simulink model "baseline_validation"  (R2024b)
settings: Solver=ode45  StartTime=0  StopTime=0.1  MaxStep=1e-4  RelTol=1e-8  AbsTol=1e-10
model workspace (MAT data in the model file):
  F = 0.008
  J = 0.003
  L = 0.0085
  Rs = 0.2
  inputFrequency = 20
  loadTorque = 0
  p = 4
  psi = 0.175
  voltageAmplitude = 30
Description:
  | AFPM 等效集中参数、非凸极 PMSM plant 独立验证；不代表三维磁场或完整闭环控制。
settings Model: Creator=m1516  LastModifiedBy=m1516
settings DataIOCC: SaveOutput=off  SignalLogging=off

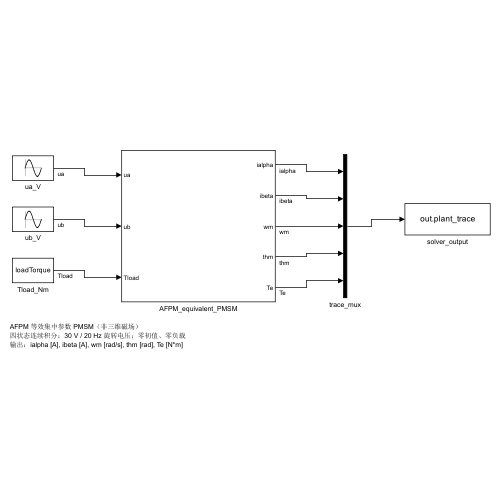
[thumbnail: Simulink's stored preview of the top-level diagram]
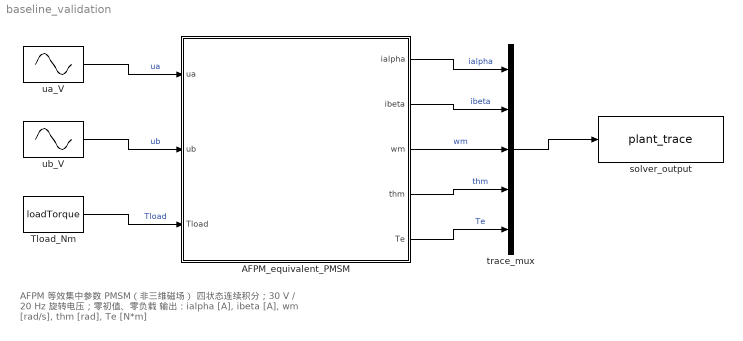
== system baseline_validation ==
  note: AFPM 等效集中参数 PMSM（非三维磁场）
      | 四状态连续积分；30 V / 20 Hz 旋转电压；零初值、零负载
      | 输出：ialpha [A], ibeta [A], wm [rad/s], thm [rad], Te [N*m]
  AFPM_equivalent_PMSM : Subsystem
  Tload_Nm : Constant  Value=loadTorque
  solver_output : ToWorkspace  VariableName=plant_trace  SaveFormat=Timeseries  SampleTime=-1
  trace_mux : Mux  Inputs=5
  ua_V : Sin  Amplitude=voltageAmplitude  Frequency=2*pi*inputFrequency  Phase=pi/2  SampleTime=0
  ub_V : Sin  Amplitude=voltageAmplitude  Frequency=2*pi*inputFrequency  SampleTime=0
  wires:
  ua_V/1 -> AFPM_equivalent_PMSM/1(ua)  "ua"
  ub_V/1 -> AFPM_equivalent_PMSM/2(ub)  "ub"
  Tload_Nm/1 -> AFPM_equivalent_PMSM/3(Tload)  "Tload"
  AFPM_equivalent_PMSM/1(ialpha) -> trace_mux/1  "ialpha"
  AFPM_equivalent_PMSM/2(ibeta) -> trace_mux/2  "ibeta"
  AFPM_equivalent_PMSM/3(wm) -> trace_mux/3  "wm"
  AFPM_equivalent_PMSM/4(thm) -> trace_mux/4  "thm"
  AFPM_equivalent_PMSM/5(Te) -> trace_mux/5  "Te"
  trace_mux/1 -> solver_output/1

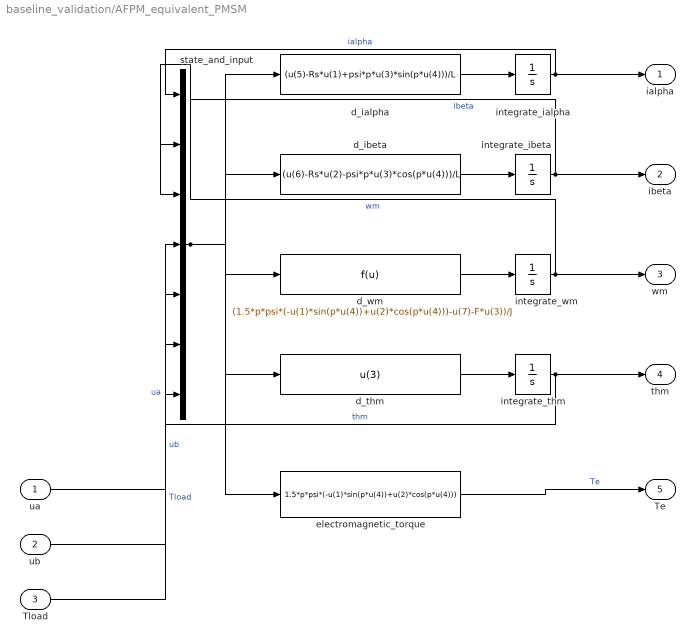
== system baseline_validation/AFPM_equivalent_PMSM ==
  ua : Inport  Unit=V
  ub : Inport  Port=2  Unit=V
  Tload : Inport  Port=3  Unit=N*m
  d_ialpha : Fcn  Expr=(u(5)-Rs*u(1)+psi*p*u(3)*sin(p*u(4)))/L
  d_ibeta : Fcn  Expr=(u(6)-Rs*u(2)-psi*p*u(3)*cos(p*u(4)))/L
  d_thm : Fcn  Expr=u(3)
  d_wm : Fcn  Expr=(1.5*p*psi*(-u(1)*sin(p*u(4))+u(2)*cos(p*u(4)))-u(7)-F*u(3))/J
  electromagnetic_torque : Fcn  Expr=1.5*p*psi*(-u(1)*sin(p*u(4))+u(2)*cos(p*u(4)))
  integrate_ialpha : Integrator
  integrate_ibeta : Integrator
  integrate_thm : Integrator
  integrate_wm : Integrator
  state_and_input : Mux  Inputs=7
  ialpha : Outport  Unit=A
  ibeta : Outport  Port=2  Unit=A
  wm : Outport  Port=3  Unit=rad/s
  thm : Outport  Port=4  Unit=rad
  Te : Outport  Port=5  Unit=N*m
  wires:
  state_and_input/1 -> d_ialpha/1, d_ibeta/1, d_wm/1, d_thm/1, electromagnetic_torque/1
  d_ialpha/1 -> integrate_ialpha/1
  integrate_ialpha/1 -> ialpha/1, state_and_input/1  "ialpha"
  d_ibeta/1 -> integrate_ibeta/1
  integrate_ibeta/1 -> ibeta/1, state_and_input/2  "ibeta"
  d_wm/1 -> integrate_wm/1
  integrate_wm/1 -> wm/1, state_and_input/3  "wm"
  d_thm/1 -> integrate_thm/1
  integrate_thm/1 -> thm/1, state_and_input/4  "thm"
  ua/1 -> state_and_input/5  "ua"
  ub/1 -> state_and_input/6  "ub"
  Tload/1 -> state_and_input/7  "Tload"
  electromagnetic_torque/1 -> Te/1  "Te"
